simulink model "analytical_models"  (R2026b)
settings: Solver=ode4  StopTime=30  FixedStep=0.003
settings Model: Creator=Thomas  LastModifiedBy=andrei
settings DataIOCC: DSMLogging=off  ReturnWorkspaceOutputs=off

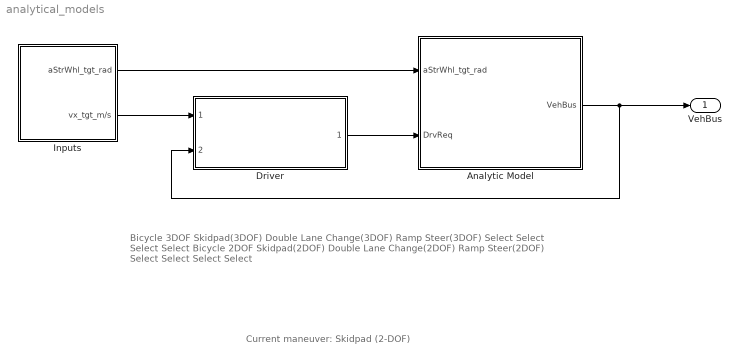
== system analytical_models ==
  note: Current maneuver: Skidpad (2-DOF)
  note: Bicycle 3DOF
      | Skidpad(3DOF)
      | Double Lane Change(3DOF)
      | Ramp Steer(3DOF)
      |
      | Select
      | Select
      | Select
      | Select
      |
      | Bicycle 2DOF
      | Skidpad(2DOF)
      | Double Lane Change(2DOF)
      | Ramp Steer(2DOF)
      |
      | Select
      | Select
      | Select
      | Select
  Analytic Model : Subsystem  Variant=on
  Driver : Subsystem  ReferencedSubsystem=Driver
  Inputs : Subsystem
  VehBus : Outport
  wires:
  Analytic Model/1(VehBus) -> Driver/2, VehBus/1
  Inputs/1(aStrWhl_tgt_rad) -> Analytic Model/1(aStrWhl_tgt_rad)
  Inputs/2(vx_tgt_m/s) -> Driver/1
  Driver/1 -> Analytic Model/2(DrvReq)

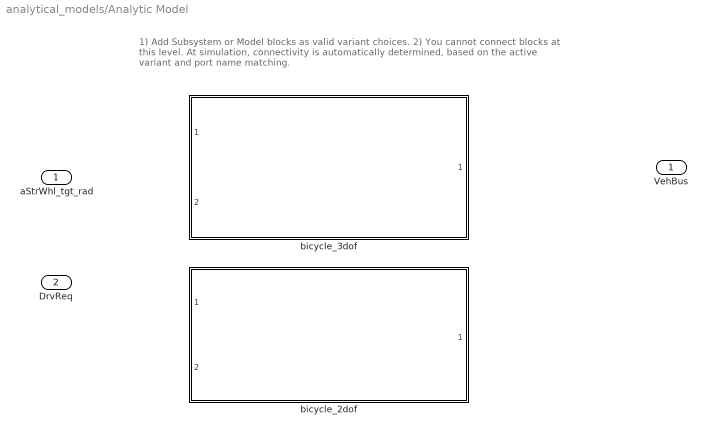
== system analytical_models/Analytic Model ==
  note: 1) Add Subsystem or Model blocks as valid variant choices.
      | 2) You cannot connect blocks at this level. At simulation, connectivity is automatically
      | determined, based on the active variant and port name matching.
  aStrWhl_tgt_rad : Inport
  DrvReq : Inport  Port=2
  bicycle_2dof : Subsystem  VariantControl=MODE==2  ReferencedSubsystem=bicycle_2dof
  bicycle_3dof : Subsystem  VariantControl=MODE==3  ReferencedSubsystem=bicycle_3dof
  VehBus : Outport

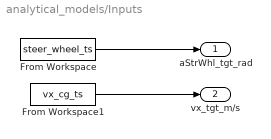
== system analytical_models/Inputs ==
  From Workspace : FromWorkspace  VariableName=steer_wheel_ts
  From Workspace1 : FromWorkspace  VariableName=vx_cg_ts
  aStrWhl_tgt_rad : Outport
  vx_tgt_m/s : Outport  Port=2
  wires:
  From Workspace1/1 -> vx_tgt_m/s/1
  From Workspace/1 -> aStrWhl_tgt_rad/1
